simulink model "SimuNolineal"  (R2026a)
settings: Solver=VariableStepAuto  StopTime=200
values from neighbouring files (symbols this model uses):
  B = 6*0.0041    (= 0.0246)    [Hinfinito.m]
  g = 9.81    [Hinfinito.m]
  I = 3.2*382.232e-7    (= 0.00012231424)    [Hinfinito.m]
  kd = 11.751    [Hinfinito.m]
  ki = 188.016    [Hinfinito.m]
  kp = 94.008    [Hinfinito.m]
  kuf = 9.2568e-04    (= 0.00092568)    [Hinfinito.m]
  lc = 40.67e-3    (= 0.04067)    [Hinfinito.m]
  m = 30.00e-3    (= 0.03)    [Hinfinito.m]
  r = 135.0e-3    (= 0.135)    [Hinfinito.m]
libraries: slpidlib x1, simulink x1
settings Model: Creator=sslan  LastModifiedBy=leonardoa29

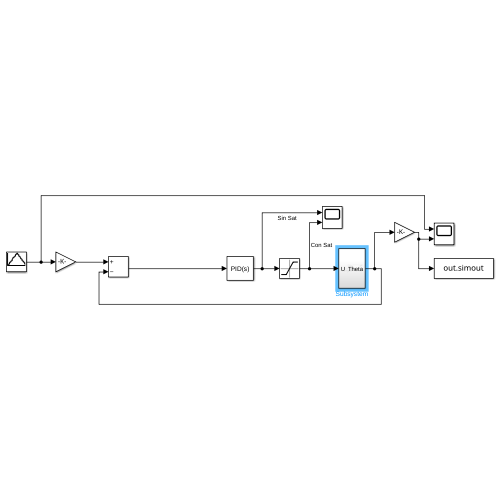
[thumbnail: Simulink's stored preview of the top-level diagram]
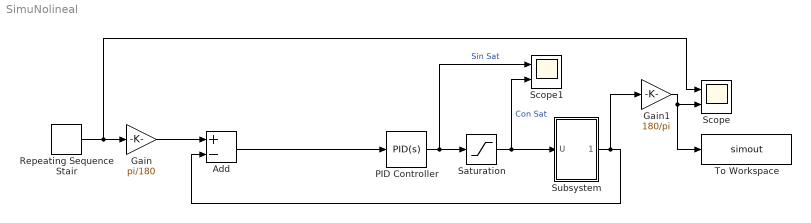
== system SimuNolineal ==
  Add : Sum  Inputs=+-
  Gain : Gain  Gain=pi/180
  Gain1 : Gain  Gain=180/pi
  PID Controller : slpidlib/PID Controller  Controller=PID  Form=Parallel  TimeDomain=Continuous-time  UseExternalTs=off  SampleTime=-1  IntegratorMethod=Forward Euler  FilterMethod=Forward Euler  ControllerParametersSource=internal  P=kp  I=ki  UseKiTs=off  D=kd  UseExternalDerivativeSource=off  N=100  UseFilter=on  TunerSelectOption=Transfer Function Based (PID Tuner App)  InitialConditionSource=internal  InitialConditionForIntegrator=0  InitialConditionForFilter=0  DifferentiatorICPrevScaledInput=0  ExternalReset=none  TrackingMode=off  Kt=1  LimitOutput=off  SatLimitsSource=internal  UpperSaturationLimit=inf  LowerSaturationLimit=-inf  LinearizeAsGain=on  AntiWindupMode=none  Kb=1  LimitIntegrator=off  UpperIntegratorSaturationLimit=inf  LowerIntegratorSaturationLimit=-inf  POutMin=[]  POutMax=[]  IOutMin=[]  IOutMax=[]  DOutMin=[]  DOutMax=[]  NOutMin=[]  NOutMax=[]  SumOutMin=[]  SumOutMax=[]  SaturationOutMin=[]  SaturationOutMax=[]  PParamMin=[]  PParamMax=[]  IParamMin=[]  IParamMax=[]  DParamMin=[]  DParamMax=[]  NParamMin=[]  NParamMax=[]  KbParamMin=[]  KbParamMax=[]  KtParamMin=[]  KtParamMax=[]  KbOutMin=[]  KbOutMax=[]  KtOutMin=[]  KtOutMax=[]  IntegratorOutMin=[]  IntegratorOutMax=[]  FilterOutMin=[]  FilterOutMax=[]  SumI1OutMin=[]  SumI1OutMax=[]  SumI2OutMin=[]  SumI2OutMax=[]  SumI3OutMin=[]  SumI3OutMax=[]  SumI4OutMin=[]  SumI4OutMax=[]  SumDOutMin=[]  SumDOutMax=[]  DifferentiatorOutMin=[]  DifferentiatorOutMax=[]  FilterDiffOutCoefMin=[]  FilterDiffOutCoefMax=[]  ReciprocalOutMin=[]  ReciprocalOutMax=[]  SumDenOutMin=[]  SumDenOutMax=[]  SumNumOutMin=[]  SumNumOutMax=[]  DivideOutMin=[]  DivideOutMax=[]  UdiffTsProdOutMin=[]  UdiffTsProdOutMax=[]  NTsProdOutMin=[]  NTsProdOutMax=[]  UintegralTsProdOutMin=[]  UintegralTsProdOutMax=[]  UngainTsProdOutMin=[]  UngainTsProdOutMax=[]  ClampingZeroOutDataTypeStr=Inherit: Inherit via back propagation  ClampingZeroOutMin=[]  ClampingZeroOutMax=[]  FilterDenConstantOutDataTypeStr=Inherit: Inherit via back propagation  FilterDenConstantOutMin=[]  FilterDenConstantOutMax=[]  PCopyOutDataTypeStr=Inherit: Inherit via back propagation  PCopyOutMin=[]  PCopyOutMax=[]  NCopyOutDataTypeStr=Inherit: Inherit via back propagation  NCopyOutMin=[]  NCopyOutMax=[]  IntegratorContinuousStateAttributes=''  IntegratorStateMustResolveToSignalObject=off  IntegratorRTWStateStorageClass=Auto  FilterContinuousStateAttributes=''  FilterStateMustResolveToSignalObject=off  FilterRTWStateStorageClass=Auto  ParallelPVariant=InternalParameters  IdealPVariant=Disabled  IVariant=InternalParameters  DVariant=InternalParameters  IntegratorVariant=Continuous  SatVariant=Disabled  AWVariant=Passthrough  PCopyVariant=Disabled  TRVariant=Disabled  FdbkBlocksVariant=Forward  IdealPFdbkVariant=Disabled  SatFdbkVariant=Disabled  DerivativeFilterVariant=ContFilter  NVariant=InternalParameters  NCopyVariant=Disabled  FilterICVariant=InternalICsFilter  IntegratorICVariant=InternalICs  ExternalResetVariant=Disabled  TRSumVariant=Passthrough  SumFdbkVariant=Disabled  SumVariant=Sum_PID  TsampFilterVariant=InternalTs  TsampNgainVariant=Passthrough  TsampIntegralVariant=Disabled_SignalSpec  ExternalSaturationOutDataTypeStr=Inherit: Same as second input  DerivativeSourceVariant=ErrorSignal  PreIntVariant=InternalPreInt
  Repeating Sequence Stair : simulink/Sources/Repeating Sequence Stair  OutValues=repeating_sequence  tsamp=step_interval  OutMin=[]  OutMax=[]  OutDataTypeStr=double  OutputDataTypeScalingMode=double  OutDataType=fixdt(0,8)  ConRadixGroup=Best Precision: Vector-wise  OutScaling=2^-12
      settings: LibrarySourceBlock=|
      | hdlsllib/Sources/Repeating
      | Sequence
      | Stair
  Saturation : Saturate  UpperLimit=100  LowerLimit=0
  Scope : Scope  NumInputPorts=2
      settings: ActiveDisplayYMinimum=-10.066002063595457  ActiveDisplayYMaximum=90.594018572359133
  Scope1 : Scope  NumInputPorts=2
      settings: ActiveDisplayYMinimum=-23185.39523  ActiveDisplayYMaximum=6141.21612  DataLoggingVariableName=ScopeData2
  Subsystem : Subsystem
  To Workspace : ToWorkspace  VariableName=simout  SaveFormat=Timeseries  SampleTime=-1
  wires:
  Subsystem/1(Theta) -> Gain1/1, Add/2
  Saturation/1 -> Scope1/2, Subsystem/1(U)  "Con Sat"
  PID Controller/1 -> Scope1/1, Saturation/1  "Sin Sat"
  Repeating Sequence Stair/1 -> Scope/1, Gain/1
  Gain/1 -> Add/1
  Gain1/1 -> To Workspace/1, Scope/2
  Add/1 -> PID Controller/1

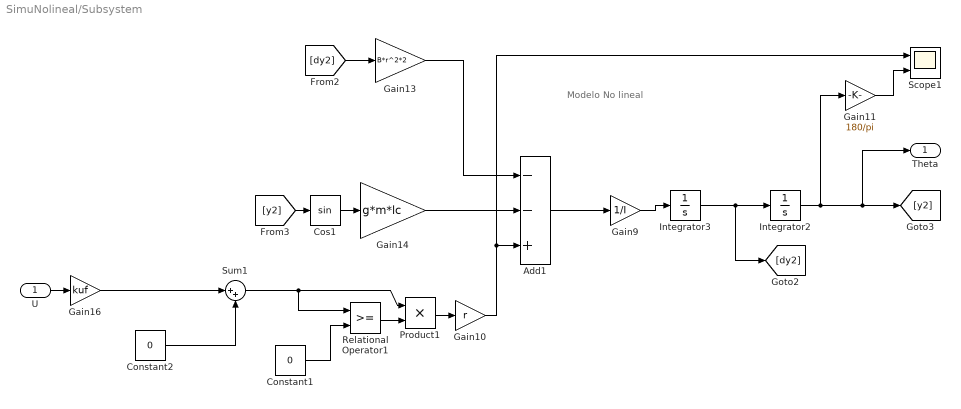
== system SimuNolineal/Subsystem ==
  note: Modelo No lineal
  U : Inport
  Add1 : Sum  Inputs=--+
  Constant1 : Constant  Value=0
  Constant2 : Constant  Value=0
  Cos1 : Trigonometry
  Gain10 : Gain  Gain=r
  Gain11 : Gain  Gain=180/pi
  Gain13 : Gain  Gain=B*r^2*2
  Gain14 : Gain  Gain=g*m*lc
  Gain16 : Gain  Gain=kuf
  Gain9 : Gain  Gain=1/I
  Integrator2 : Integrator
  Integrator3 : Integrator
  Product1 : Product
  Relational Operator1 : RelationalOperator  OutDataTypeStr=boolean  RndMeth=Simplest  InputSameDT=off
  Scope1 : Scope  NumInputPorts=2
      settings: ActiveDisplayYMinimum=-6.18885  ActiveDisplayYMaximum=55.69963
  Sum1 : Sum  Inputs=|++
  Theta : Outport
  wires:
  Integrator2/1 -> Theta/1, [y2], Gain11/1
  [y2] -> Cos1/1
  Constant1/1 -> Relational Operator1/2
  Gain10/1 -> Add1/3, Scope1/1
  Relational Operator1/1 -> Product1/2
  Sum1/1 -> Product1/1, Relational Operator1/1
  Gain11/1 -> Scope1/2
  [dy2] -> Gain13/1
  Constant2/1 -> Sum1/2
  Gain14/1 -> Add1/2
  Gain13/1 -> Add1/1
  Gain16/1 -> Sum1/1
  Add1/1 -> Gain9/1
  Gain9/1 -> Integrator3/1
  Cos1/1 -> Gain14/1
  Integrator3/1 -> [dy2], Integrator2/1
  Product1/1 -> Gain10/1
  U/1 -> Gain16/1
